simulink model "MLI17"  (R2025a)
settings: Solver=ode45  StartTime=0.0  StopTime=.5  RelTol=1e-3  EnableMultiTasking=on
libraries: spsMosfetLib x12, spsSeriesRLCBranchLib x11, spsVoltageMeasurementLib x10, spsDiodeLib x8, spsControlledCurrentSourceLib x8, spsCurrentMeasurementLib x8, spsParallelRLCLoadLib x1, spspowerguiLib x1
(part 1 of 2)
settings Model: SimulationMode=accelerator  Creator=Indhu  LastModifiedBy=SimuVerity Contributors
settings SolverCC: AlgebraicLoopSolver=TrustRegion
settings DataIOCC: LimitDataPoints=on  SaveFormat=Array  ReturnWorkspaceOutputs=off
settings OptimizationCC: ExpressionDepthLimit=2147483647.0  LifeSpan=inf
settings DebuggingCC: UnderspecifiedInitializationDetection=Classic  MergeDetectMultiDrivingBlocksExec=none  SolverPrmCheckMsg=warning  UnconnectedInputMsg=warning  UnconnectedOutputMsg=warning  UnconnectedLineMsg=warning  StateNameClashWarn=warning  SFUnexpectedBacktrackingDiag=warning  SFNoUnconditionalDefaultTransitionDiag=warning  SFExecutionAtInitializationDiag=none  ArithmeticOperatorsInVariantConditions=warning
settings HardwareCC: ProdBitPerPointer=32.0  ProdBitPerSizeT=32.0  ProdBitPerPtrDiffT=32.0  ProdLargestAtomicFloat=None  ProdIntDivRoundTo=Undefined  ProdEndianess=Unspecified  ProdWordSize=32.0  ProdHWDeviceType=32-bit Generic
settings ModelReferenceCC: PropagateSignalLabelsOutOfModel=off
settings SFSimCC: SimUseLocalCustomCode=off  CustomCodeUndefinedFunction=UseInterfaceOnly
settings RTWCC: RTWUseLocalCustomCode=off  GPUComputeCapability=3.5
settings CodeAppCC: StateflowObjectComments=on
settings GRTTargetCC: TargetLangStandard=C89/C90 (ANSI)
settings ConfigComp: CovMetricSettings=dw  CovSaveCumulativeToWorkspaceVar=on  CovSaveSingleToWorkspaceVar=on  CovExternalEMLEnable=off
settings SimscapeCC: SimscapeNormalizeSystem=off

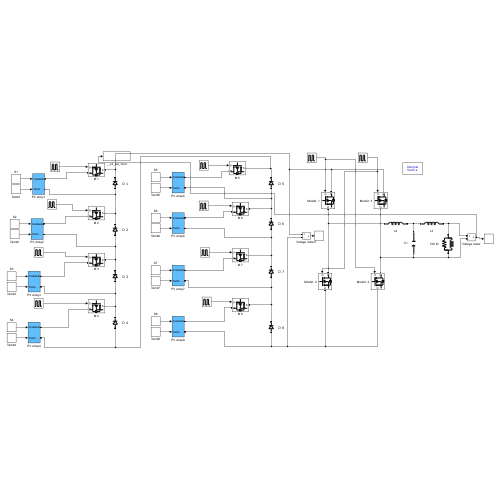
[thumbnail: Simulink's stored preview of the top-level diagram]
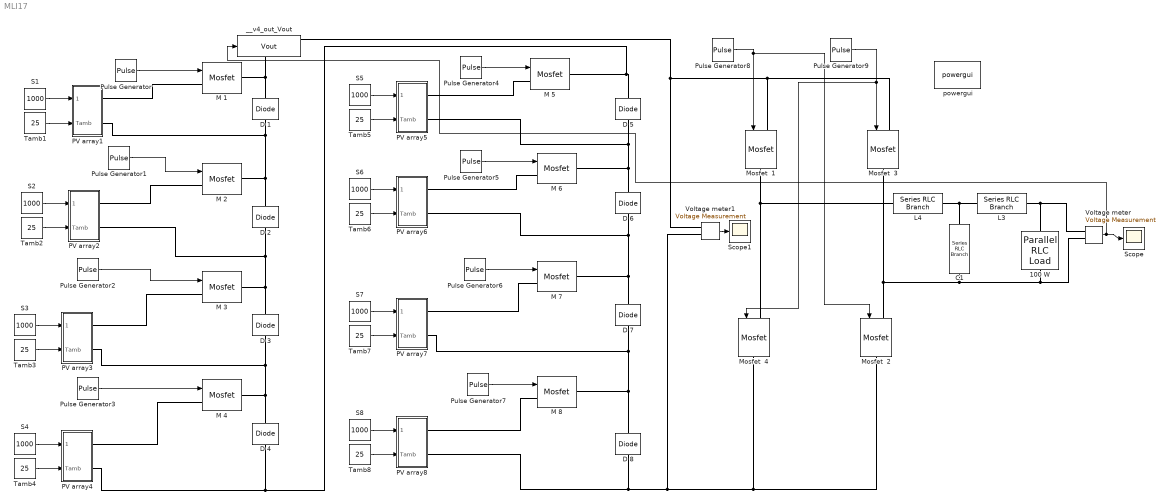
== system MLI17 ==
  100 W : spsParallelRLCLoadLib/Parallel RLC Load  LConnTagsString=a  RConnTagsString=__new0  NominalVoltage=230  NominalFrequency=50  ActivePower=P_load  InductivePower=1  CapacitivePower=0  Setx0=off  InitialVoltage=0  SetiL0=off  InitialCurrent=0  Measurements=None  LoadType=constant Z
      settings: AttributesFormatString=\n  LibrarySourceBlock=sps_lib/Passives/Parallel RLC Load
  C1 : spsSeriesRLCBranchLib/Series RLC Branch  LConnTagsString=__new0  RConnTagsString=__new0  BranchType=C  Resistance=1  Inductance=1e-3  SetiL0=off  InitialCurrent=0  Capacitance=15.5e-5  Setx0=off  InitialVoltage=0  Measurements=None
  D {1..8} (8 alike) : spsDiodeLib/Diode  Ron=0.00001  Lon=0  Vf=0  IC=0  UseSnubber=off  Rs=inf  Cs=0  Measurements=off
  L3 : spsSeriesRLCBranchLib/Series RLC Branch  LConnTagsString=__new0  RConnTagsString=__new0  BranchType=L  Resistance=1  Inductance=0.0499  SetiL0=off  InitialCurrent=0  Capacitance=1e-6  Setx0=off  InitialVoltage=0  Measurements=None
  L4 : spsSeriesRLCBranchLib/Series RLC Branch  LConnTagsString=__new0  RConnTagsString=__new0  BranchType=L  Resistance=1  Inductance=0.04999  SetiL0=off  InitialCurrent=0  Capacitance=1e-6  Setx0=off  InitialVoltage=0  Measurements=None
  M {1..8} (8 alike) : spsMosfetLib/Mosfet  Ron=0.1  Lon=0  Rd=0.01  Vfd=0  IC=0  Rs=1e5  Cs=inf  Measurements=off
  Mosfet  {1..4} (4 alike) : spsMosfetLib/Mosfet  Ron=0.1  Lon=0  Rd=0.01  Vfd=0  IC=0  Rs=1e5  Cs=inf  Measurements=off
  PV array1 : Subsystem
  PV array2 : Subsystem
  PV array3 : Subsystem
  PV array4 : Subsystem
  PV array5 : Subsystem
  PV array6 : Subsystem
  PV array7 : Subsystem
  PV array8 : Subsystem
  Pulse Generator : DiscretePulseGenerator  PulseType=Time based  Period=0.01  PulseWidth=99.999  VectorParams1D=off
  Pulse Generator1 : DiscretePulseGenerator  PulseType=Time based  Period=0.01  PulseWidth=87.5  PhaseDelay=0.000625
  Pulse Generator2 : DiscretePulseGenerator  PulseType=Time based  Period=0.01  PulseWidth=75  PhaseDelay=0.00125
  Pulse Generator3 : DiscretePulseGenerator  PulseType=Time based  Period=0.01  PulseWidth=62.5  PhaseDelay=0.001875
  Pulse Generator4 : DiscretePulseGenerator  PulseType=Time based  Period=0.01  PulseWidth=50  PhaseDelay=0.0025
  Pulse Generator5 : DiscretePulseGenerator  PulseType=Time based  Period=0.01  PulseWidth=37.5  PhaseDelay=0.003125
  Pulse Generator6 : DiscretePulseGenerator  PulseType=Time based  Period=0.01  PulseWidth=25  PhaseDelay=0.00375
  Pulse Generator7 : DiscretePulseGenerator  PulseType=Time based  Period=0.01  PulseWidth=12.5  PhaseDelay=0.004375
  Pulse Generator8 : DiscretePulseGenerator  PulseType=Time based  Period=0.02  PulseWidth=50
  Pulse Generator9 : DiscretePulseGenerator  PulseType=Time based  Period=0.02  PulseWidth=50  PhaseDelay=0.01
  S{1..8} (8 alike) : Constant  Value=1000
  Scope : Scope
      settings: RequirementInfo="{}  %GIDa_4b453156_1c3c_43c0_866a_e0860ec2177e"  Title=17 level output voltage for MCI with LCL filter  ActiveDisplayYMinimum=-225  ActiveDisplayYMaximum=225  DataLoggingMaxPoints=500000000  DataLoggingVariableName=ML
  Scope1 : Scope
      settings: Title="Multilevel DC-DC  output Voltage waveform"
  Tamb{1..8} (8 alike) : Constant  Value=25
  Voltage meter : spsVoltageMeasurementLib/Voltage Measurement  PhasorSimulation=off  OutputType=Complex  PSBequivalent=0
  Voltage meter1 : spsVoltageMeasurementLib/Voltage Measurement  PhasorSimulation=off  OutputType=Complex  PSBequivalent=0
  __v4_out_Vout : ToWorkspace  VariableName=Vout  SaveFormat=Timeseries  SampleTime=-1
  powergui : spspowerguiLib/powergui  Priority=1  SimulationMode=Discrete  SampleTime=50e-6  frequency=60  Iterations=50  frequencyindice=0  Pbase=100e6  ErrMax=1e-4  UnitsV=kV  UnitsW=MW  buscounter=0  FunctionMessages=off  echomessages=off  EnableUseOfTLC=off  CurrentSourceSwitches=off  DisableSnubberDevices=off  DisableRonSwitches=off  DisableVfSwitches=off  DisplayEquations=off  AutomaticDiscreteSolvers=off  SolverType=Tustin  Interpol=off  ExternalGateDelay=off  methode=off  Ts=100  x0status=blocks  SPID=off  SwTol=0  HookPort=off  NonlinearTolerance=1e-4  nMaxIteration=100  ContinueOnMaxIteration=off  RestoreLinks=warning  ResistiveCurrentMeasurement=off  Frange=[0:2:500]  Ylog=off  Xlog=on  ShowGrid=off  save=off  variable=ZData  structure=ML  ZoomFFT=off  StartTime=0.15  cycles=10  DisplayStyle=1  fundamental=50  FreqAxis=off  MaxFrequency=1000  frequencyindicesteady=1  RmsSteady=1  display=off
  wires:
  Voltage meter/1 -> Scope/1, __v4_out_Vout/1
  Pulse Generator/1 -> M 1/1
  Pulse Generator1/1 -> M 2/1
  Pulse Generator2/1 -> M 3/1
  Pulse Generator3/1 -> M 4/1
  Pulse Generator4/1 -> M 5/1
  Pulse Generator5/1 -> M 6/1
  Pulse Generator6/1 -> M 7/1
  Pulse Generator7/1 -> M 8/1
  Pulse Generator8/1 -> Mosfet  2/1, Mosfet  1/1
  Pulse Generator9/1 -> Mosfet  4/1, Mosfet  3/1
  Voltage meter1/1 -> Scope1/1
  Tamb1/1 -> PV array1/2(Tamb)
  S1/1 -> PV array1/1(irradiance)
  Tamb2/1 -> PV array2/2(Tamb)
  S2/1 -> PV array2/1(irradiance)
  Tamb3/1 -> PV array3/2(Tamb)
  S3/1 -> PV array3/1(irradiance)
  Tamb4/1 -> PV array4/2(Tamb)
  S4/1 -> PV array4/1(irradiance)
  Tamb5/1 -> PV array5/2(Tamb)
  S5/1 -> PV array5/1(irradiance)
  Tamb6/1 -> PV array6/2(Tamb)
  S6/1 -> PV array6/1(irradiance)
  Tamb7/1 -> PV array7/2(Tamb)
  S7/1 -> PV array7/1(irradiance)
  Tamb8/1 -> PV array8/2(Tamb)
  S8/1 -> PV array8/1(irradiance)
  connections:
  M 1/LConn1 -- PV array1/RConn1
  D 1/LConn1 -- D 2/RConn1 -- M 2/RConn1 -- PV array1/RConn2
  D 2/LConn1 -- PV array2/RConn2 -- D 3/RConn1 -- M 3/RConn1
  D 3/LConn1 -- D 4/RConn1 -- M 4/RConn1 -- PV array3/RConn2
  M 8/RConn1 -- D 8/RConn1 -- D 7/LConn1 -- PV array7/RConn2
  D 6/LConn1 -- PV array6/RConn2 -- D 7/RConn1 -- M 7/RConn1
  M 6/RConn1 -- D 6/RConn1 -- PV array5/RConn2 -- D 5/LConn1
  M 2/LConn1 -- PV array2/RConn1
  M 3/LConn1 -- PV array3/RConn1
  M 4/LConn1 -- PV array4/RConn1
  D 4/LConn1 -- PV array4/RConn2 -- D 5/RConn1 -- M 5/RConn1
  M 5/LConn1 -- PV array5/RConn1
  M 6/LConn1 -- PV array6/RConn1
  M 7/LConn1 -- PV array7/RConn1
  M 8/LConn1 -- PV array8/RConn1
  Mosfet  4/LConn1 -- L4/LConn1 -- Mosfet  1/RConn1
  Mosfet  3/RConn1 -- C1/RConn1 -- 100 W/RConn1 -- Voltage meter/LConn2 -- Mosfet  2/LConn1
  Voltage meter1/LConn2 -- Mosfet  2/RConn1 -- Mosfet  4/RConn1 -- PV array8/RConn2 -- D 8/LConn1
  Mosfet  1/LConn1 -- Mosfet  3/LConn1 -- Voltage meter1/LConn1 -- M 1/RConn1 -- D 1/RConn1
  C1/LConn1 -- L3/LConn1 -- L4/RConn1
  100 W/LConn1 -- Voltage meter/LConn1 -- L3/RConn1

== system MLI17/PV array1 ==
  irradiance : Inport
  Tamb : Inport  Port=2
  4700uF : spsSeriesRLCBranchLib/Series RLC Branch  LConnTagsString=__new0  RConnTagsString=__new0  BranchType=C  Resistance=1  Inductance=5e-03  SetiL0=off  InitialCurrent=0  Capacitance=4700e-6  Setx0=off  InitialVoltage=0  Measurements=None
  CCS : spsControlledCurrentSourceLib/Controlled Current Source  Initialize=on  Source_Type=AC  Amplitude=0  Phase=0  Frequency=0  Measurements=None
  CM : spsCurrentMeasurementLib/Current Measurement  PhasorSimulation=off  OutputType=Complex  PSBequivalent=0
  Im : Constant  Value=10
  Isc : Constant  Value=12
  Saturation : Saturate  UpperLimit=100  LowerLimit=0
  Saturation1 : Saturate  UpperLimit=4  LowerLimit=0
  Subsystem1 : Subsystem
  Tref : Constant  Value=55
  VM1 : spsVoltageMeasurementLib/Voltage Measurement  PhasorSimulation=off  OutputType=Complex  PSBequivalent=0
  Vm : Constant  Value=28
  Voc : Constant  Value=28.75
  + : PMIOPort  Tag=PMCPort  Side=Right
  - : PMIOPort  Tag=PMCPort  Port=2  Side=Right
  wires:
  Isc/1 -> Subsystem1/4(Isc)
  Im/1 -> Subsystem1/6(Im)
  Voc/1 -> Subsystem1/5(Voc)
  Vm/1 -> Subsystem1/7(Vm)
  irradiance/1 -> Subsystem1/2(S)
  Tamb/1 -> Subsystem1/3(Tamb)
  Saturation/1 -> Subsystem1/1(Vpv)
  VM1/1 -> Saturation/1
  Tref/1 -> Subsystem1/8(Tref)
  Subsystem1/1(Ipv) -> Saturation1/1
  Saturation1/1 -> CCS/1
  connections:
  CCS/RConn1 -- CM/LConn1
  +/RConn1 -- CM/RConn1 -- VM1/LConn1 -- 4700uF/LConn1
  -/RConn1 -- CCS/LConn1 -- VM1/LConn2 -- 4700uF/RConn1

== system MLI17/PV array2 ==
  irradiance : Inport
  Tamb : Inport  Port=2
  4700uF : spsSeriesRLCBranchLib/Series RLC Branch  LConnTagsString=__new0  RConnTagsString=__new0  BranchType=C  Resistance=1  Inductance=5e-03  SetiL0=off  InitialCurrent=0  Capacitance=4700e-6  Setx0=off  InitialVoltage=0  Measurements=None
  CCS : spsControlledCurrentSourceLib/Controlled Current Source  Initialize=on  Source_Type=AC  Amplitude=0  Phase=0  Frequency=0  Measurements=None
  CM : spsCurrentMeasurementLib/Current Measurement  PhasorSimulation=off  OutputType=Complex  PSBequivalent=0
  Im : Constant  Value=10
  Isc : Constant  Value=12
  Saturation : Saturate  UpperLimit=100  LowerLimit=0
  Saturation1 : Saturate  UpperLimit=4  LowerLimit=0
  Subsystem1 : Subsystem
  Tref : Constant  Value=55
  VM1 : spsVoltageMeasurementLib/Voltage Measurement  PhasorSimulation=off  OutputType=Complex  PSBequivalent=0
  Vm : Constant  Value=28
  Voc : Constant  Value=28.75
  + : PMIOPort  Tag=PMCPort  Side=Right
  - : PMIOPort  Tag=PMCPort  Port=2  Side=Right
  wires:
  Saturation1/1 -> CCS/1
  Subsystem1/1(Ipv) -> Saturation1/1
  Tref/1 -> Subsystem1/8(Tref)
  VM1/1 -> Saturation/1
  Saturation/1 -> Subsystem1/1(Vpv)
  Tamb/1 -> Subsystem1/3(Tamb)
  irradiance/1 -> Subsystem1/2(S)
  Vm/1 -> Subsystem1/7(Vm)
  Voc/1 -> Subsystem1/5(Voc)
  Im/1 -> Subsystem1/6(Im)
  Isc/1 -> Subsystem1/4(Isc)
  connections:
  4700uF/RConn1 -- VM1/LConn2 -- CCS/LConn1 -- -/RConn1
  4700uF/LConn1 -- VM1/LConn1 -- CM/RConn1 -- +/RConn1
  CCS/RConn1 -- CM/LConn1

== system MLI17/PV array3 ==
  irradiance : Inport
  Tamb : Inport  Port=2
  4700uF : spsSeriesRLCBranchLib/Series RLC Branch  LConnTagsString=__new0  RConnTagsString=__new0  BranchType=C  Resistance=1  Inductance=5e-03  SetiL0=off  InitialCurrent=0  Capacitance=4700e-6  Setx0=off  InitialVoltage=0  Measurements=None
  CCS : spsControlledCurrentSourceLib/Controlled Current Source  Initialize=on  Source_Type=AC  Amplitude=0  Phase=0  Frequency=0  Measurements=None
  CM : spsCurrentMeasurementLib/Current Measurement  PhasorSimulation=off  OutputType=Complex  PSBequivalent=0
  Im : Constant  Value=10
  Isc : Constant  Value=12
  Saturation : Saturate  UpperLimit=100  LowerLimit=0
  Saturation1 : Saturate  UpperLimit=4  LowerLimit=0
  Subsystem1 : Subsystem
  Tref : Constant  Value=55
  VM1 : spsVoltageMeasurementLib/Voltage Measurement  PhasorSimulation=off  OutputType=Complex  PSBequivalent=0
  Vm : Constant  Value=28
  Voc : Constant  Value=28.75
  + : PMIOPort  Tag=PMCPort  Side=Right
  - : PMIOPort  Tag=PMCPort  Port=2  Side=Right
  wires:
  Isc/1 -> Subsystem1/4(Isc)
  Im/1 -> Subsystem1/6(Im)
  Voc/1 -> Subsystem1/5(Voc)
  Vm/1 -> Subsystem1/7(Vm)
  irradiance/1 -> Subsystem1/2(S)
  Tamb/1 -> Subsystem1/3(Tamb)
  Saturation/1 -> Subsystem1/1(Vpv)
  VM1/1 -> Saturation/1
  Tref/1 -> Subsystem1/8(Tref)
  Subsystem1/1(Ipv) -> Saturation1/1
  Saturation1/1 -> CCS/1
  connections:
  CCS/RConn1 -- CM/LConn1
  +/RConn1 -- CM/RConn1 -- VM1/LConn1 -- 4700uF/LConn1
  -/RConn1 -- CCS/LConn1 -- VM1/LConn2 -- 4700uF/RConn1

== system MLI17/PV array4 ==
  irradiance : Inport
  Tamb : Inport  Port=2
  4700uF : spsSeriesRLCBranchLib/Series RLC Branch  LConnTagsString=__new0  RConnTagsString=__new0  BranchType=C  Resistance=1  Inductance=5e-03  SetiL0=off  InitialCurrent=0  Capacitance=4700e-6  Setx0=off  InitialVoltage=0  Measurements=None
  CCS : spsControlledCurrentSourceLib/Controlled Current Source  Initialize=on  Source_Type=AC  Amplitude=0  Phase=0  Frequency=0  Measurements=None
  CM : spsCurrentMeasurementLib/Current Measurement  PhasorSimulation=off  OutputType=Complex  PSBequivalent=0
  Im : Constant  Value=10
  Isc : Constant  Value=12
  Saturation : Saturate  UpperLimit=100  LowerLimit=0
  Saturation1 : Saturate  UpperLimit=4  LowerLimit=0
  Subsystem1 : Subsystem
  Tref : Constant  Value=55
  VM1 : spsVoltageMeasurementLib/Voltage Measurement  PhasorSimulation=off  OutputType=Complex  PSBequivalent=0
  Vm : Constant  Value=28
  Voc : Constant  Value=28.75
  + : PMIOPort  Tag=PMCPort  Side=Right
  - : PMIOPort  Tag=PMCPort  Port=2  Side=Right
  wires:
  Saturation1/1 -> CCS/1
  Subsystem1/1(Ipv) -> Saturation1/1
  Tref/1 -> Subsystem1/8(Tref)
  VM1/1 -> Saturation/1
  Saturation/1 -> Subsystem1/1(Vpv)
  Tamb/1 -> Subsystem1/3(Tamb)
  irradiance/1 -> Subsystem1/2(S)
  Vm/1 -> Subsystem1/7(Vm)
  Voc/1 -> Subsystem1/5(Voc)
  Im/1 -> Subsystem1/6(Im)
  Isc/1 -> Subsystem1/4(Isc)
  connections:
  4700uF/RConn1 -- VM1/LConn2 -- CCS/LConn1 -- -/RConn1
  4700uF/LConn1 -- VM1/LConn1 -- CM/RConn1 -- +/RConn1
  CCS/RConn1 -- CM/LConn1

== system MLI17/PV array5 ==
  irradiance : Inport
  Tamb : Inport  Port=2
  4700uF : spsSeriesRLCBranchLib/Series RLC Branch  LConnTagsString=__new0  RConnTagsString=__new0  BranchType=C  Resistance=1  Inductance=5e-03  SetiL0=off  InitialCurrent=0  Capacitance=4700e-6  Setx0=off  InitialVoltage=0  Measurements=None
  CCS : spsControlledCurrentSourceLib/Controlled Current Source  Initialize=on  Source_Type=AC  Amplitude=0  Phase=0  Frequency=0  Measurements=None
  CM : spsCurrentMeasurementLib/Current Measurement  PhasorSimulation=off  OutputType=Complex  PSBequivalent=0
  Im : Constant  Value=10
  Isc : Constant  Value=12
  Saturation : Saturate  UpperLimit=100  LowerLimit=0
  Saturation1 : Saturate  UpperLimit=4  LowerLimit=0
  Subsystem1 : Subsystem
  Tref : Constant  Value=55
  VM1 : spsVoltageMeasurementLib/Voltage Measurement  PhasorSimulation=off  OutputType=Complex  PSBequivalent=0
  Vm : Constant  Value=28
  Voc : Constant  Value=28.75
  + : PMIOPort  Tag=PMCPort  Side=Right
  - : PMIOPort  Tag=PMCPort  Port=2  Side=Right
  wires:
  Isc/1 -> Subsystem1/4(Isc)
  Im/1 -> Subsystem1/6(Im)
  Voc/1 -> Subsystem1/5(Voc)
  Vm/1 -> Subsystem1/7(Vm)
  irradiance/1 -> Subsystem1/2(S)
  Tamb/1 -> Subsystem1/3(Tamb)
  Saturation/1 -> Subsystem1/1(Vpv)
  VM1/1 -> Saturation/1
  Tref/1 -> Subsystem1/8(Tref)
  Subsystem1/1(Ipv) -> Saturation1/1
  Saturation1/1 -> CCS/1
  connections:
  CCS/RConn1 -- CM/LConn1
  +/RConn1 -- CM/RConn1 -- VM1/LConn1 -- 4700uF/LConn1
  -/RConn1 -- CCS/LConn1 -- VM1/LConn2 -- 4700uF/RConn1

== system MLI17/PV array6 ==
  irradiance : Inport
  Tamb : Inport  Port=2
  4700uF : spsSeriesRLCBranchLib/Series RLC Branch  LConnTagsString=__new0  RConnTagsString=__new0  BranchType=C  Resistance=1  Inductance=5e-03  SetiL0=off  InitialCurrent=0  Capacitance=4700e-6  Setx0=off  InitialVoltage=0  Measurements=None
  CCS : spsControlledCurrentSourceLib/Controlled Current Source  Initialize=on  Source_Type=AC  Amplitude=0  Phase=0  Frequency=0  Measurements=None
  CM : spsCurrentMeasurementLib/Current Measurement  PhasorSimulation=off  OutputType=Complex  PSBequivalent=0
  Im : Constant  Value=10
  Isc : Constant  Value=12
  Saturation : Saturate  UpperLimit=100  LowerLimit=0
  Saturation1 : Saturate  UpperLimit=4  LowerLimit=0
  Subsystem1 : Subsystem
  Tref : Constant  Value=55
  VM1 : spsVoltageMeasurementLib/Voltage Measurement  PhasorSimulation=off  OutputType=Complex  PSBequivalent=0
  Vm : Constant  Value=28
  Voc : Constant  Value=28.75
  + : PMIOPort  Tag=PMCPort  Side=Right
  - : PMIOPort  Tag=PMCPort  Port=2  Side=Right
  wires:
  Saturation1/1 -> CCS/1
  Subsystem1/1(Ipv) -> Saturation1/1
  Tref/1 -> Subsystem1/8(Tref)
  VM1/1 -> Saturation/1
  Saturation/1 -> Subsystem1/1(Vpv)
  Tamb/1 -> Subsystem1/3(Tamb)
  irradiance/1 -> Subsystem1/2(S)
  Vm/1 -> Subsystem1/7(Vm)
  Voc/1 -> Subsystem1/5(Voc)
  Im/1 -> Subsystem1/6(Im)
  Isc/1 -> Subsystem1/4(Isc)
  connections:
  4700uF/RConn1 -- VM1/LConn2 -- CCS/LConn1 -- -/RConn1
  4700uF/LConn1 -- VM1/LConn1 -- CM/RConn1 -- +/RConn1
  CCS/RConn1 -- CM/LConn1

== system MLI17/PV array7 ==
  irradiance : Inport
  Tamb : Inport  Port=2
  4700uF : spsSeriesRLCBranchLib/Series RLC Branch  LConnTagsString=__new0  RConnTagsString=__new0  BranchType=C  Resistance=1  Inductance=5e-03  SetiL0=off  InitialCurrent=0  Capacitance=4700e-6  Setx0=off  InitialVoltage=0  Measurements=None
  CCS : spsControlledCurrentSourceLib/Controlled Current Source  Initialize=on  Source_Type=AC  Amplitude=0  Phase=0  Frequency=0  Measurements=None
  CM : spsCurrentMeasurementLib/Current Measurement  PhasorSimulation=off  OutputType=Complex  PSBequivalent=0
  Im : Constant  Value=10
  Isc : Constant  Value=12
  Saturation : Saturate  UpperLimit=100  LowerLimit=0
  Saturation1 : Saturate  UpperLimit=4  LowerLimit=0
  Subsystem1 : Subsystem
  Tref : Constant  Value=55
  VM1 : spsVoltageMeasurementLib/Voltage Measurement  PhasorSimulation=off  OutputType=Complex  PSBequivalent=0
  Vm : Constant  Value=28
  Voc : Constant  Value=28.75
  + : PMIOPort  Tag=PMCPort  Side=Right
  - : PMIOPort  Tag=PMCPort  Port=2  Side=Right
  wires:
  Isc/1 -> Subsystem1/4(Isc)
  Im/1 -> Subsystem1/6(Im)
  Voc/1 -> Subsystem1/5(Voc)
  Vm/1 -> Subsystem1/7(Vm)
  irradiance/1 -> Subsystem1/2(S)
  Tamb/1 -> Subsystem1/3(Tamb)
  Saturation/1 -> Subsystem1/1(Vpv)
  VM1/1 -> Saturation/1
  Tref/1 -> Subsystem1/8(Tref)
  Subsystem1/1(Ipv) -> Saturation1/1
  Saturation1/1 -> CCS/1
  connections:
  CCS/RConn1 -- CM/LConn1
  +/RConn1 -- CM/RConn1 -- VM1/LConn1 -- 4700uF/LConn1
  -/RConn1 -- CCS/LConn1 -- VM1/LConn2 -- 4700uF/RConn1

== system MLI17/PV array8 ==
  irradiance : Inport
  Tamb : Inport  Port=2
  4700uF : spsSeriesRLCBranchLib/Series RLC Branch  LConnTagsString=__new0  RConnTagsString=__new0  BranchType=C  Resistance=1  Inductance=5e-03  SetiL0=off  InitialCurrent=0  Capacitance=4700e-6  Setx0=off  InitialVoltage=0  Measurements=None
  CCS : spsControlledCurrentSourceLib/Controlled Current Source  Initialize=on  Source_Type=AC  Amplitude=0  Phase=0  Frequency=0  Measurements=None
  CM : spsCurrentMeasurementLib/Current Measurement  PhasorSimulation=off  OutputType=Complex  PSBequivalent=0
  Im : Constant  Value=10
  Isc : Constant  Value=12
  Saturation : Saturate  UpperLimit=100  LowerLimit=0
  Saturation1 : Saturate  UpperLimit=4  LowerLimit=0
  Subsystem1 : Subsystem
  Tref : Constant  Value=55
  VM1 : spsVoltageMeasurementLib/Voltage Measurement  PhasorSimulation=off  OutputType=Complex  PSBequivalent=0
  Vm : Constant  Value=28
  Voc : Constant  Value=28.75
  + : PMIOPort  Tag=PMCPort  Side=Right
  - : PMIOPort  Tag=PMCPort  Port=2  Side=Right
  wires:
  Saturation1/1 -> CCS/1
  Subsystem1/1(Ipv) -> Saturation1/1
  Tref/1 -> Subsystem1/8(Tref)
  VM1/1 -> Saturation/1
  Saturation/1 -> Subsystem1/1(Vpv)
  Tamb/1 -> Subsystem1/3(Tamb)
  irradiance/1 -> Subsystem1/2(S)
  Vm/1 -> Subsystem1/7(Vm)
  Voc/1 -> Subsystem1/5(Voc)
  Im/1 -> Subsystem1/6(Im)
  Isc/1 -> Subsystem1/4(Isc)
  connections:
  4700uF/RConn1 -- VM1/LConn2 -- CCS/LConn1 -- -/RConn1
  4700uF/LConn1 -- VM1/LConn1 -- CM/RConn1 -- +/RConn1
  CCS/RConn1 -- CM/LConn1

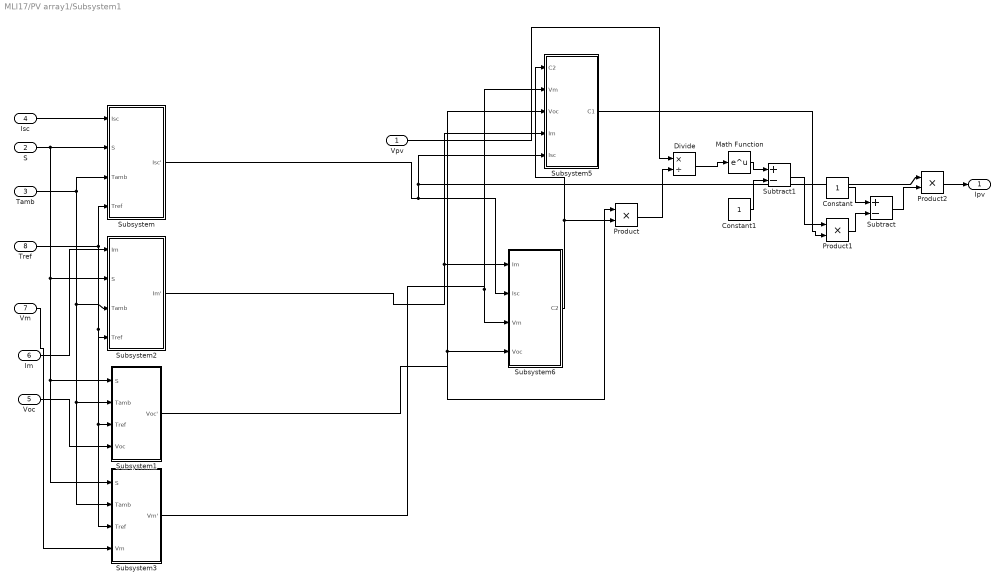
== system MLI17/PV array1/Subsystem1 ==
  Vpv : Inport
  S : Inport  Port=2
  Tamb : Inport  Port=3
  Isc : Inport  Port=4
  Voc : Inport  Port=5
  Im : Inport  Port=6
  Vm : Inport  Port=7
  Tref : Inport  Port=8
  Constant : Constant
  Constant1 : Constant
  Divide : Product  Inputs=*/
  Math Function : Math  SignedPower=on
  Product : Product  RndMeth=Zero
  Product1 : Product  RndMeth=Zero
  Product2 : Product  RndMeth=Zero
  Subsystem : Subsystem
  Subsystem1 : Subsystem
  Subsystem2 : Subsystem
  Subsystem3 : Subsystem
  Subsystem5 : Subsystem
  Subsystem6 : Subsystem
  Subtract : Sum  Inputs=+-
  Subtract1 : Sum  Inputs=+-
  Ipv : Outport
  wires:
  Product/1 -> Divide/2
  Constant/1 -> Subtract/1
  Product1/1 -> Subtract/2
  Subtract/1 -> Product2/2
  Product2/1 -> Ipv/1
  Divide/1 -> Math Function/1
  Math Function/1 -> Subtract1/1
  Constant1/1 -> Subtract1/2
  Subtract1/1 -> Product1/1
  Subsystem2/1(Im') -> Subsystem6/1(Im), Subsystem5/4(Im)
  Subsystem/1(Isc') -> Subsystem6/2(Isc), Product2/1, Subsystem5/5(Isc)
  Subsystem1/1(Voc') -> Product/1, Subsystem5/3(Voc), Subsystem6/4(Voc)
  Subsystem3/1(Vm') -> Subsystem5/2(Vm), Subsystem6/3(Vm)
  Subsystem6/1(C2) -> Subsystem5/1(C2), Product/2
  Vpv/1 -> Divide/1
  Subsystem5/1(C1) -> Product1/2
  Isc/1 -> Subsystem/1(Isc)
  S/1 -> Subsystem1/1(S), Subsystem3/1(S), Subsystem2/2(S), Subsystem/2(S)
  Tamb/1 -> Subsystem1/2(Tamb), Subsystem3/2(Tamb), Subsystem2/3(Tamb), Subsystem/3(Tamb)
  Tref/1 -> Subsystem1/3(Tref), Subsystem3/3(Tref), Subsystem2/4(Tref), Subsystem/4(Tref)
  Im/1 -> Subsystem2/1(Im)
  Voc/1 -> Subsystem1/4(Voc)
  Vm/1 -> Subsystem3/4(Vm)

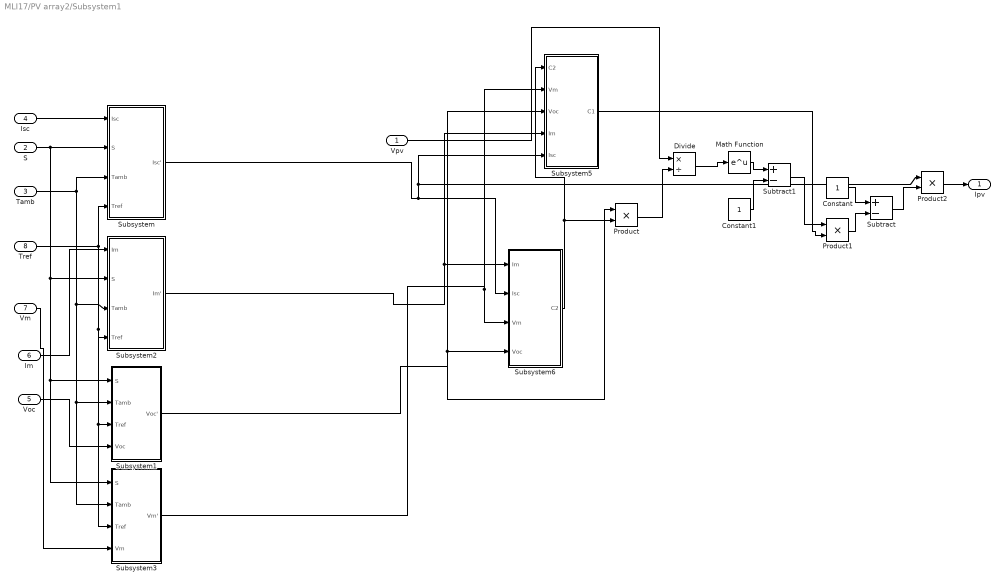
== system MLI17/PV array2/Subsystem1 ==
  Vpv : Inport
  S : Inport  Port=2
  Tamb : Inport  Port=3
  Isc : Inport  Port=4
  Voc : Inport  Port=5
  Im : Inport  Port=6
  Vm : Inport  Port=7
  Tref : Inport  Port=8
  Constant : Constant
  Constant1 : Constant
  Divide : Product  Inputs=*/
  Math Function : Math  SignedPower=on
  Product : Product  RndMeth=Zero
  Product1 : Product  RndMeth=Zero
  Product2 : Product  RndMeth=Zero
  Subsystem : Subsystem
  Subsystem1 : Subsystem
  Subsystem2 : Subsystem
  Subsystem3 : Subsystem
  Subsystem5 : Subsystem
  Subsystem6 : Subsystem
  Subtract : Sum  Inputs=+-
  Subtract1 : Sum  Inputs=+-
  Ipv : Outport
  wires:
  Vm/1 -> Subsystem3/4(Vm)
  Voc/1 -> Subsystem1/4(Voc)
  Im/1 -> Subsystem2/1(Im)
  Tref/1 -> Subsystem/4(Tref), Subsystem2/4(Tref), Subsystem3/3(Tref), Subsystem1/3(Tref)
  Tamb/1 -> Subsystem/3(Tamb), Subsystem2/3(Tamb), Subsystem3/2(Tamb), Subsystem1/2(Tamb)
  S/1 -> Subsystem/2(S), Subsystem2/2(S), Subsystem3/1(S), Subsystem1/1(S)
  Isc/1 -> Subsystem/1(Isc)
  Subsystem5/1(C1) -> Product1/2
  Vpv/1 -> Divide/1
  Subsystem6/1(C2) -> Product/2, Subsystem5/1(C2)
  Subsystem3/1(Vm') -> Subsystem6/3(Vm), Subsystem5/2(Vm)
  Subsystem1/1(Voc') -> Subsystem6/4(Voc), Subsystem5/3(Voc), Product/1
  Subsystem/1(Isc') -> Subsystem5/5(Isc), Product2/1, Subsystem6/2(Isc)
  Subsystem2/1(Im') -> Subsystem5/4(Im), Subsystem6/1(Im)
  Subtract1/1 -> Product1/1
  Constant1/1 -> Subtract1/2
  Math Function/1 -> Subtract1/1
  Divide/1 -> Math Function/1
  Product2/1 -> Ipv/1
  Subtract/1 -> Product2/2
  Product1/1 -> Subtract/2
  Constant/1 -> Subtract/1
  Product/1 -> Divide/2

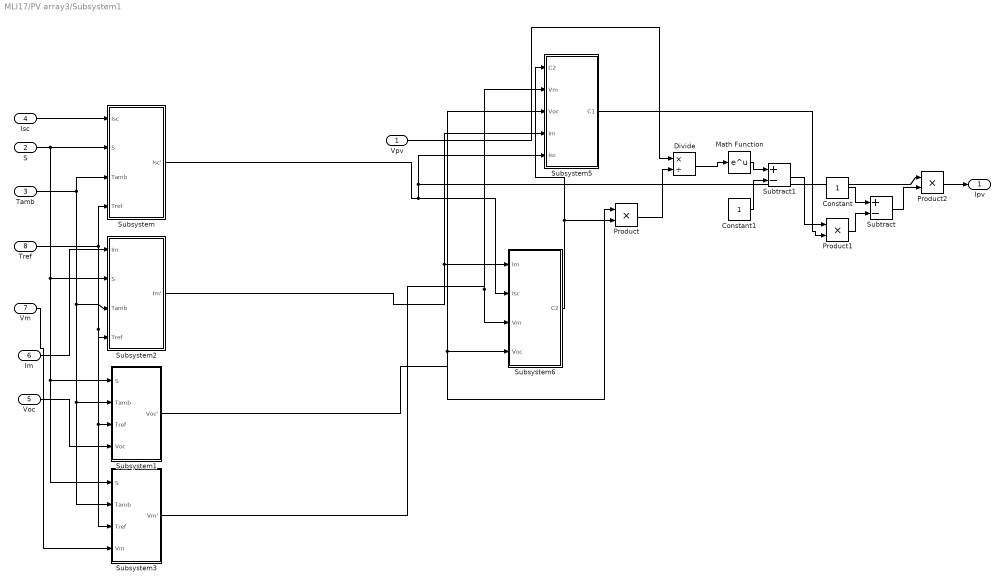
== system MLI17/PV array3/Subsystem1 ==
  Vpv : Inport
  S : Inport  Port=2
  Tamb : Inport  Port=3
  Isc : Inport  Port=4
  Voc : Inport  Port=5
  Im : Inport  Port=6
  Vm : Inport  Port=7
  Tref : Inport  Port=8
  Constant : Constant
  Constant1 : Constant
  Divide : Product  Inputs=*/
  Math Function : Math  SignedPower=on
  Product : Product  RndMeth=Zero
  Product1 : Product  RndMeth=Zero
  Product2 : Product  RndMeth=Zero
  Subsystem : Subsystem
  Subsystem1 : Subsystem
  Subsystem2 : Subsystem
  Subsystem3 : Subsystem
  Subsystem5 : Subsystem
  Subsystem6 : Subsystem
  Subtract : Sum  Inputs=+-
  Subtract1 : Sum  Inputs=+-
  Ipv : Outport
  wires:
  Product/1 -> Divide/2
  Constant/1 -> Subtract/1
  Product1/1 -> Subtract/2
  Subtract/1 -> Product2/2
  Product2/1 -> Ipv/1
  Divide/1 -> Math Function/1
  Math Function/1 -> Subtract1/1
  Constant1/1 -> Subtract1/2
  Subtract1/1 -> Product1/1
  Subsystem2/1(Im') -> Subsystem6/1(Im), Subsystem5/4(Im)
  Subsystem/1(Isc') -> Subsystem6/2(Isc), Product2/1, Subsystem5/5(Isc)
  Subsystem1/1(Voc') -> Product/1, Subsystem5/3(Voc), Subsystem6/4(Voc)
  Subsystem3/1(Vm') -> Subsystem5/2(Vm), Subsystem6/3(Vm)
  Subsystem6/1(C2) -> Subsystem5/1(C2), Product/2
  Vpv/1 -> Divide/1
  Subsystem5/1(C1) -> Product1/2
  Isc/1 -> Subsystem/1(Isc)
  S/1 -> Subsystem1/1(S), Subsystem3/1(S), Subsystem2/2(S), Subsystem/2(S)
  Tamb/1 -> Subsystem1/2(Tamb), Subsystem3/2(Tamb), Subsystem2/3(Tamb), Subsystem/3(Tamb)
  Tref/1 -> Subsystem1/3(Tref), Subsystem3/3(Tref), Subsystem2/4(Tref), Subsystem/4(Tref)
  Im/1 -> Subsystem2/1(Im)
  Voc/1 -> Subsystem1/4(Voc)
  Vm/1 -> Subsystem3/4(Vm)

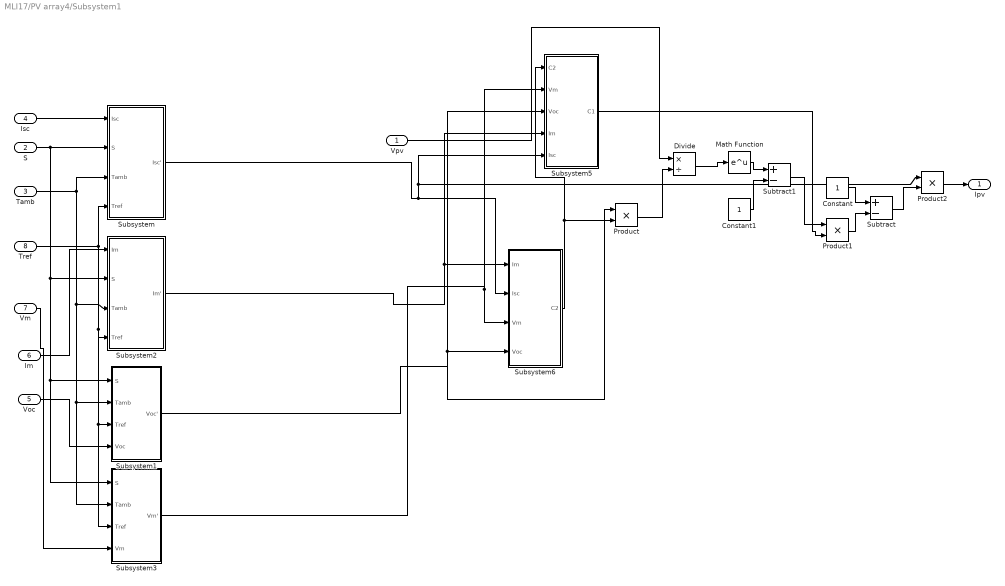
== system MLI17/PV array4/Subsystem1 ==
  Vpv : Inport
  S : Inport  Port=2
  Tamb : Inport  Port=3
  Isc : Inport  Port=4
  Voc : Inport  Port=5
  Im : Inport  Port=6
  Vm : Inport  Port=7
  Tref : Inport  Port=8
  Constant : Constant
  Constant1 : Constant
  Divide : Product  Inputs=*/
  Math Function : Math  SignedPower=on
  Product : Product  RndMeth=Zero
  Product1 : Product  RndMeth=Zero
  Product2 : Product  RndMeth=Zero
  Subsystem : Subsystem
  Subsystem1 : Subsystem
  Subsystem2 : Subsystem
  Subsystem3 : Subsystem
  Subsystem5 : Subsystem
  Subsystem6 : Subsystem
  Subtract : Sum  Inputs=+-
  Subtract1 : Sum  Inputs=+-
  Ipv : Outport
  wires:
  Vm/1 -> Subsystem3/4(Vm)
  Voc/1 -> Subsystem1/4(Voc)
  Im/1 -> Subsystem2/1(Im)
  Tref/1 -> Subsystem/4(Tref), Subsystem2/4(Tref), Subsystem3/3(Tref), Subsystem1/3(Tref)
  Tamb/1 -> Subsystem/3(Tamb), Subsystem2/3(Tamb), Subsystem3/2(Tamb), Subsystem1/2(Tamb)
  S/1 -> Subsystem/2(S), Subsystem2/2(S), Subsystem3/1(S), Subsystem1/1(S)
  Isc/1 -> Subsystem/1(Isc)
  Subsystem5/1(C1) -> Product1/2
  Vpv/1 -> Divide/1
  Subsystem6/1(C2) -> Product/2, Subsystem5/1(C2)
  Subsystem3/1(Vm') -> Subsystem6/3(Vm), Subsystem5/2(Vm)
  Subsystem1/1(Voc') -> Subsystem6/4(Voc), Subsystem5/3(Voc), Product/1
  Subsystem/1(Isc') -> Subsystem5/5(Isc), Product2/1, Subsystem6/2(Isc)
  Subsystem2/1(Im') -> Subsystem5/4(Im), Subsystem6/1(Im)
  Subtract1/1 -> Product1/1
  Constant1/1 -> Subtract1/2
  Math Function/1 -> Subtract1/1
  Divide/1 -> Math Function/1
  Product2/1 -> Ipv/1
  Subtract/1 -> Product2/2
  Product1/1 -> Subtract/2
  Constant/1 -> Subtract/1
  Product/1 -> Divide/2

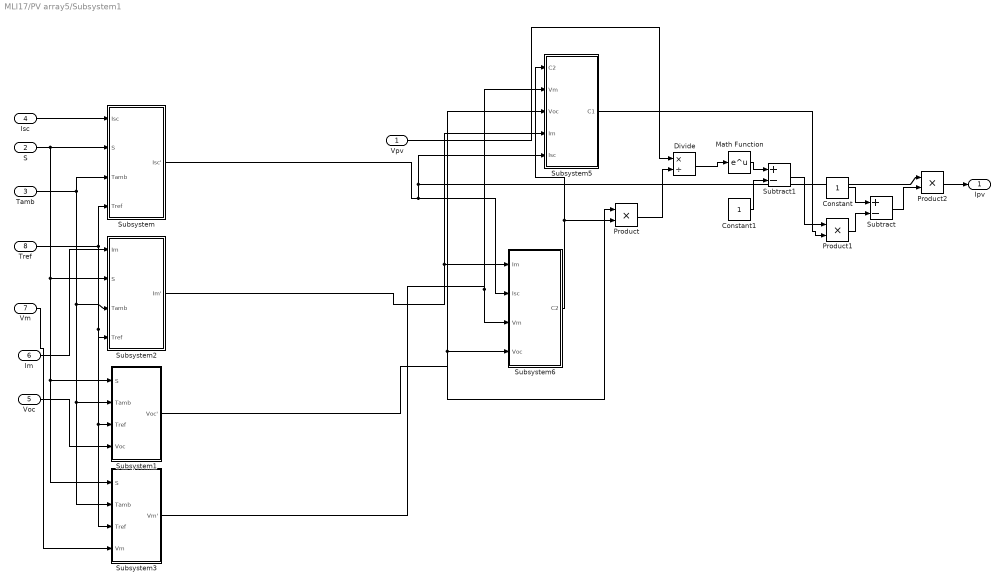
== system MLI17/PV array5/Subsystem1 ==
  Vpv : Inport
  S : Inport  Port=2
  Tamb : Inport  Port=3
  Isc : Inport  Port=4
  Voc : Inport  Port=5
  Im : Inport  Port=6
  Vm : Inport  Port=7
  Tref : Inport  Port=8
  Constant : Constant
  Constant1 : Constant
  Divide : Product  Inputs=*/
  Math Function : Math  SignedPower=on
  Product : Product  RndMeth=Zero
  Product1 : Product  RndMeth=Zero
  Product2 : Product  RndMeth=Zero
  Subsystem : Subsystem
  Subsystem1 : Subsystem
  Subsystem2 : Subsystem
  Subsystem3 : Subsystem
  Subsystem5 : Subsystem
  Subsystem6 : Subsystem
  Subtract : Sum  Inputs=+-
  Subtract1 : Sum  Inputs=+-
  Ipv : Outport
  wires:
  Product/1 -> Divide/2
  Constant/1 -> Subtract/1
  Product1/1 -> Subtract/2
  Subtract/1 -> Product2/2
  Product2/1 -> Ipv/1
  Divide/1 -> Math Function/1
  Math Function/1 -> Subtract1/1
  Constant1/1 -> Subtract1/2
  Subtract1/1 -> Product1/1
  Subsystem2/1(Im') -> Subsystem6/1(Im), Subsystem5/4(Im)
  Subsystem/1(Isc') -> Subsystem6/2(Isc), Product2/1, Subsystem5/5(Isc)
  Subsystem1/1(Voc') -> Product/1, Subsystem5/3(Voc), Subsystem6/4(Voc)
  Subsystem3/1(Vm') -> Subsystem5/2(Vm), Subsystem6/3(Vm)
  Subsystem6/1(C2) -> Subsystem5/1(C2), Product/2
  Vpv/1 -> Divide/1
  Subsystem5/1(C1) -> Product1/2
  Isc/1 -> Subsystem/1(Isc)
  S/1 -> Subsystem1/1(S), Subsystem3/1(S), Subsystem2/2(S), Subsystem/2(S)
  Tamb/1 -> Subsystem1/2(Tamb), Subsystem3/2(Tamb), Subsystem2/3(Tamb), Subsystem/3(Tamb)
  Tref/1 -> Subsystem1/3(Tref), Subsystem3/3(Tref), Subsystem2/4(Tref), Subsystem/4(Tref)
  Im/1 -> Subsystem2/1(Im)
  Voc/1 -> Subsystem1/4(Voc)
  Vm/1 -> Subsystem3/4(Vm)

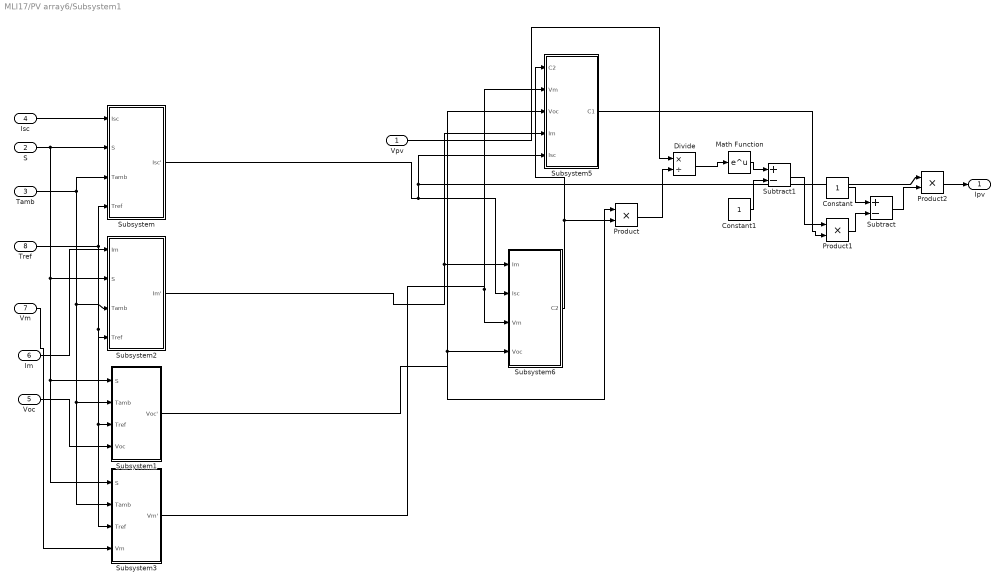
== system MLI17/PV array6/Subsystem1 ==
  Vpv : Inport
  S : Inport  Port=2
  Tamb : Inport  Port=3
  Isc : Inport  Port=4
  Voc : Inport  Port=5
  Im : Inport  Port=6
  Vm : Inport  Port=7
  Tref : Inport  Port=8
  Constant : Constant
  Constant1 : Constant
  Divide : Product  Inputs=*/
  Math Function : Math  SignedPower=on
  Product : Product  RndMeth=Zero
  Product1 : Product  RndMeth=Zero
  Product2 : Product  RndMeth=Zero
  Subsystem : Subsystem
  Subsystem1 : Subsystem
  Subsystem2 : Subsystem
  Subsystem3 : Subsystem
  Subsystem5 : Subsystem
  Subsystem6 : Subsystem
  Subtract : Sum  Inputs=+-
  Subtract1 : Sum  Inputs=+-
  Ipv : Outport
  wires:
  Vm/1 -> Subsystem3/4(Vm)
  Voc/1 -> Subsystem1/4(Voc)
  Im/1 -> Subsystem2/1(Im)
  Tref/1 -> Subsystem/4(Tref), Subsystem2/4(Tref), Subsystem3/3(Tref), Subsystem1/3(Tref)
  Tamb/1 -> Subsystem/3(Tamb), Subsystem2/3(Tamb), Subsystem3/2(Tamb), Subsystem1/2(Tamb)
  S/1 -> Subsystem/2(S), Subsystem2/2(S), Subsystem3/1(S), Subsystem1/1(S)
  Isc/1 -> Subsystem/1(Isc)
  Subsystem5/1(C1) -> Product1/2
  Vpv/1 -> Divide/1
  Subsystem6/1(C2) -> Product/2, Subsystem5/1(C2)
  Subsystem3/1(Vm') -> Subsystem6/3(Vm), Subsystem5/2(Vm)
  Subsystem1/1(Voc') -> Subsystem6/4(Voc), Subsystem5/3(Voc), Product/1
  Subsystem/1(Isc') -> Subsystem5/5(Isc), Product2/1, Subsystem6/2(Isc)
  Subsystem2/1(Im') -> Subsystem5/4(Im), Subsystem6/1(Im)
  Subtract1/1 -> Product1/1
  Constant1/1 -> Subtract1/2
  Math Function/1 -> Subtract1/1
  Divide/1 -> Math Function/1
  Product2/1 -> Ipv/1
  Subtract/1 -> Product2/2
  Product1/1 -> Subtract/2
  Constant/1 -> Subtract/1
  Product/1 -> Divide/2

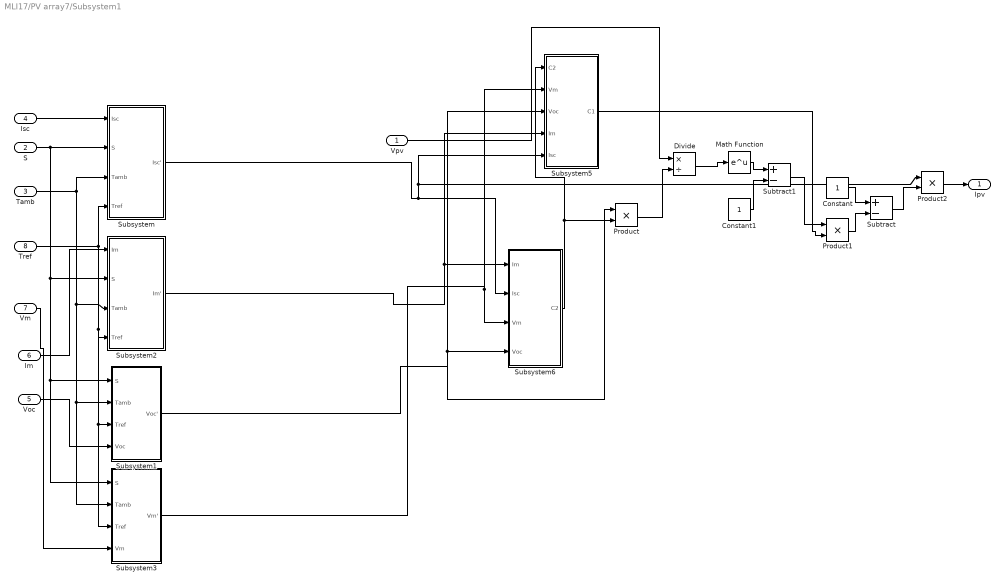
== system MLI17/PV array7/Subsystem1 ==
  Vpv : Inport
  S : Inport  Port=2
  Tamb : Inport  Port=3
  Isc : Inport  Port=4
  Voc : Inport  Port=5
  Im : Inport  Port=6
  Vm : Inport  Port=7
  Tref : Inport  Port=8
  Constant : Constant
  Constant1 : Constant
  Divide : Product  Inputs=*/
  Math Function : Math  SignedPower=on
  Product : Product  RndMeth=Zero
  Product1 : Product  RndMeth=Zero
  Product2 : Product  RndMeth=Zero
  Subsystem : Subsystem
  Subsystem1 : Subsystem
  Subsystem2 : Subsystem
  Subsystem3 : Subsystem
  Subsystem5 : Subsystem
  Subsystem6 : Subsystem
  Subtract : Sum  Inputs=+-
  Subtract1 : Sum  Inputs=+-
  Ipv : Outport
  wires:
  Product/1 -> Divide/2
  Constant/1 -> Subtract/1
  Product1/1 -> Subtract/2
  Subtract/1 -> Product2/2
  Product2/1 -> Ipv/1
  Divide/1 -> Math Function/1
  Math Function/1 -> Subtract1/1
  Constant1/1 -> Subtract1/2
  Subtract1/1 -> Product1/1
  Subsystem2/1(Im') -> Subsystem6/1(Im), Subsystem5/4(Im)
  Subsystem/1(Isc') -> Subsystem6/2(Isc), Product2/1, Subsystem5/5(Isc)
  Subsystem1/1(Voc') -> Product/1, Subsystem5/3(Voc), Subsystem6/4(Voc)
  Subsystem3/1(Vm') -> Subsystem5/2(Vm), Subsystem6/3(Vm)
  Subsystem6/1(C2) -> Subsystem5/1(C2), Product/2
  Vpv/1 -> Divide/1
  Subsystem5/1(C1) -> Product1/2
  Isc/1 -> Subsystem/1(Isc)
  S/1 -> Subsystem1/1(S), Subsystem3/1(S), Subsystem2/2(S), Subsystem/2(S)
  Tamb/1 -> Subsystem1/2(Tamb), Subsystem3/2(Tamb), Subsystem2/3(Tamb), Subsystem/3(Tamb)
  Tref/1 -> Subsystem1/3(Tref), Subsystem3/3(Tref), Subsystem2/4(Tref), Subsystem/4(Tref)
  Im/1 -> Subsystem2/1(Im)
  Voc/1 -> Subsystem1/4(Voc)
  Vm/1 -> Subsystem3/4(Vm)

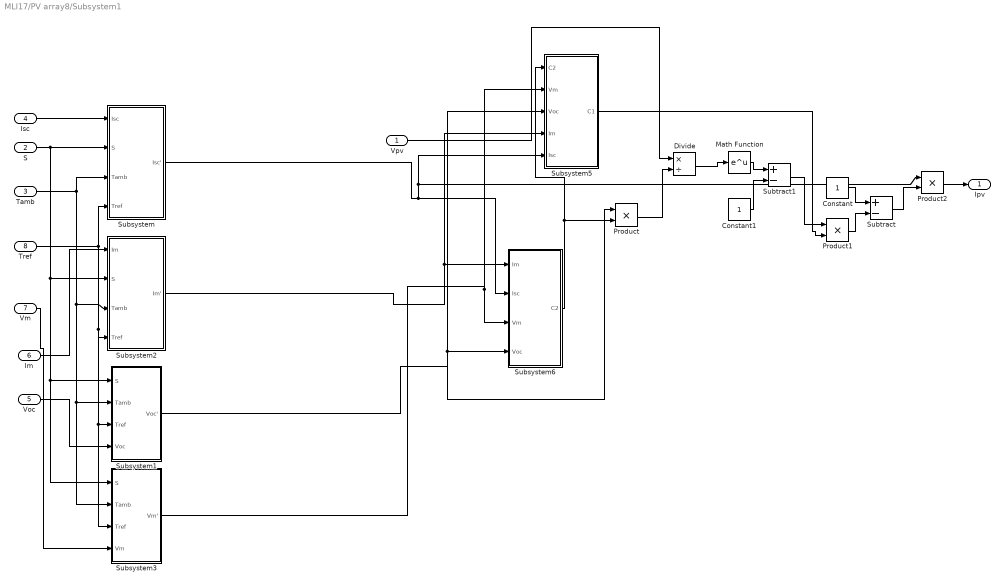
== system MLI17/PV array8/Subsystem1 ==
  Vpv : Inport
  S : Inport  Port=2
  Tamb : Inport  Port=3
  Isc : Inport  Port=4
  Voc : Inport  Port=5
  Im : Inport  Port=6
  Vm : Inport  Port=7
  Tref : Inport  Port=8
  Constant : Constant
  Constant1 : Constant
  Divide : Product  Inputs=*/
  Math Function : Math  SignedPower=on
  Product : Product  RndMeth=Zero
  Product1 : Product  RndMeth=Zero
  Product2 : Product  RndMeth=Zero
  Subsystem : Subsystem
  Subsystem1 : Subsystem
  Subsystem2 : Subsystem
  Subsystem3 : Subsystem
  Subsystem5 : Subsystem
  Subsystem6 : Subsystem
  Subtract : Sum  Inputs=+-
  Subtract1 : Sum  Inputs=+-
  Ipv : Outport
  wires:
  Vm/1 -> Subsystem3/4(Vm)
  Voc/1 -> Subsystem1/4(Voc)
  Im/1 -> Subsystem2/1(Im)
  Tref/1 -> Subsystem/4(Tref), Subsystem2/4(Tref), Subsystem3/3(Tref), Subsystem1/3(Tref)
  Tamb/1 -> Subsystem/3(Tamb), Subsystem2/3(Tamb), Subsystem3/2(Tamb), Subsystem1/2(Tamb)
  S/1 -> Subsystem/2(S), Subsystem2/2(S), Subsystem3/1(S), Subsystem1/1(S)
  Isc/1 -> Subsystem/1(Isc)
  Subsystem5/1(C1) -> Product1/2
  Vpv/1 -> Divide/1
  Subsystem6/1(C2) -> Product/2, Subsystem5/1(C2)
  Subsystem3/1(Vm') -> Subsystem6/3(Vm), Subsystem5/2(Vm)
  Subsystem1/1(Voc') -> Subsystem6/4(Voc), Subsystem5/3(Voc), Product/1
  Subsystem/1(Isc') -> Subsystem5/5(Isc), Product2/1, Subsystem6/2(Isc)
  Subsystem2/1(Im') -> Subsystem5/4(Im), Subsystem6/1(Im)
  Subtract1/1 -> Product1/1
  Constant1/1 -> Subtract1/2
  Math Function/1 -> Subtract1/1
  Divide/1 -> Math Function/1
  Product2/1 -> Ipv/1
  Subtract/1 -> Product2/2
  Product1/1 -> Subtract/2
  Constant/1 -> Subtract/1
  Product/1 -> Divide/2

== system MLI17/PV array1/Subsystem1/Subsystem ==
  Isc : Inport
  S : Inport  Port=2
  Tamb : Inport  Port=3
  Tref : Inport  Port=4
  Add : Sum
  Add1 : Sum
  Constant1 : Constant
  Constant2 : Constant  Value=0.03
  Divide : Product  Inputs=*/
  Product{,1..3} (4 alike) : Product  RndMeth=Zero
  Sref : Constant  Value=1000
  Subtract : Sum  Inputs=+-
  a : Constant  Value=0.0025
  Isc' : Outport
  wires:
  Subtract/1 -> Product/2
  a/1 -> Product/1
  Constant1/1 -> Add/2
  Product/1 -> Add/1
  Isc/1 -> Product1/1
  S/1 -> Product1/2, Product3/1
  Product1/1 -> Product2/1
  Add/1 -> Product2/2
  Product2/1 -> Divide/1
  Sref/1 -> Divide/2
  Divide/1 -> Isc'/1
  Tref/1 -> Subtract/2
  Constant2/1 -> Product3/2
  Product3/1 -> Add1/1
  Tamb/1 -> Add1/2
  Add1/1 -> Subtract/1

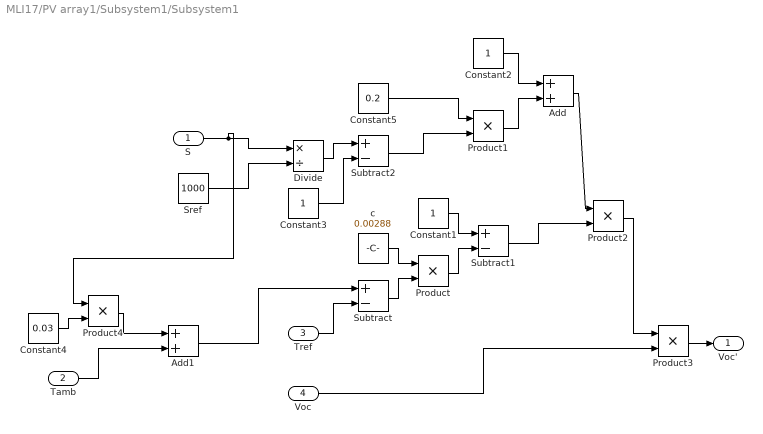
== system MLI17/PV array1/Subsystem1/Subsystem1 ==
  S : Inport
  Tamb : Inport  Port=2
  Tref : Inport  Port=3
  Voc : Inport  Port=4
  Add : Sum
  Add1 : Sum
  Constant1 : Constant
  Constant2 : Constant
  Constant3 : Constant
  Constant4 : Constant  Value=0.03
  Constant5 : Constant  Value=0.2
  Divide : Product  Inputs=*/
  Product{,1..4} (5 alike) : Product  RndMeth=Zero
  Sref : Constant  Value=1000
  Subtract : Sum  Inputs=+-
  Subtract1 : Sum  Inputs=+-
  Subtract2 : Sum  Inputs=+-
  c : Constant  Value=0.00288
  Voc' : Outport
  wires:
  Tref/1 -> Subtract/2
  c/1 -> Product/1
  Subtract/1 -> Product/2
  Constant1/1 -> Subtract1/1
  Product/1 -> Subtract1/2
  Subtract2/1 -> Product1/2
  Constant2/1 -> Add/1
  Product1/1 -> Add/2
  Subtract1/1 -> Product2/2
  Add/1 -> Product2/1
  Product2/1 -> Product3/1
  Voc/1 -> Product3/2
  Product3/1 -> Voc'/1
  S/1 -> Divide/1, Product4/1
  Sref/1 -> Divide/2
  Divide/1 -> Subtract2/1
  Constant3/1 -> Subtract2/2
  Constant4/1 -> Product4/2
  Product4/1 -> Add1/1
  Tamb/1 -> Add1/2
  Add1/1 -> Subtract/1
  Constant5/1 -> Product1/1

== system MLI17/PV array1/Subsystem1/Subsystem2 ==
  Im : Inport
  S : Inport  Port=2
  Tamb : Inport  Port=3
  Tref : Inport  Port=4
  Add : Sum
  Add1 : Sum
  Constant1 : Constant
  Constant2 : Constant  Value=0.03
  Divide : Product  Inputs=*/
  Product{,1..3} (4 alike) : Product  RndMeth=Zero
  Sref : Constant  Value=1000
  Subtract : Sum  Inputs=+-
  a : Constant  Value=0.0025
  Im' : Outport
  wires:
  Subtract/1 -> Product/2
  a/1 -> Product/1
  Constant1/1 -> Add/2
  Product/1 -> Add/1
  Im/1 -> Product1/1
  S/1 -> Product1/2, Product3/1
  Product1/1 -> Product2/1
  Add/1 -> Product2/2
  Product2/1 -> Divide/1
  Sref/1 -> Divide/2
  Divide/1 -> Im'/1
  Tref/1 -> Subtract/2
  Constant2/1 -> Product3/2
  Product3/1 -> Add1/1
  Tamb/1 -> Add1/2
  Add1/1 -> Subtract/1

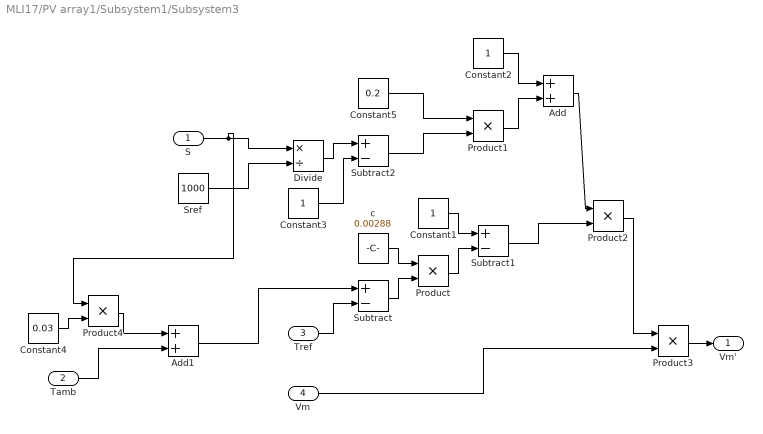
== system MLI17/PV array1/Subsystem1/Subsystem3 ==
  S : Inport
  Tamb : Inport  Port=2
  Tref : Inport  Port=3
  Vm : Inport  Port=4
  Add : Sum
  Add1 : Sum
  Constant1 : Constant
  Constant2 : Constant
  Constant3 : Constant
  Constant4 : Constant  Value=0.03
  Constant5 : Constant  Value=0.2
  Divide : Product  Inputs=*/
  Product{,1..4} (5 alike) : Product  RndMeth=Zero
  Sref : Constant  Value=1000
  Subtract : Sum  Inputs=+-
  Subtract1 : Sum  Inputs=+-
  Subtract2 : Sum  Inputs=+-
  c : Constant  Value=0.00288
  Vm' : Outport
  wires:
  Tref/1 -> Subtract/2
  c/1 -> Product/1
  Subtract/1 -> Product/2
  Constant1/1 -> Subtract1/1
  Product/1 -> Subtract1/2
  Subtract2/1 -> Product1/2
  Constant2/1 -> Add/1
  Product1/1 -> Add/2
  Subtract1/1 -> Product2/2
  Add/1 -> Product2/1
  Product2/1 -> Product3/1
  Vm/1 -> Product3/2
  Product3/1 -> Vm'/1
  S/1 -> Divide/1, Product4/1
  Sref/1 -> Divide/2
  Divide/1 -> Subtract2/1
  Constant3/1 -> Subtract2/2
  Constant4/1 -> Product4/2
  Product4/1 -> Add1/1
  Tamb/1 -> Add1/2
  Add1/1 -> Subtract/1
  Constant5/1 -> Product1/1

== system MLI17/PV array1/Subsystem1/Subsystem5 ==
  C2 : Inport
  Vm : Inport  Port=2
  Voc : Inport  Port=3
  Im : Inport  Port=4
  Isc : Inport  Port=5
  Constant : Constant
  Constant1 : Constant  Value=-1
  Divide : Product  Inputs=*/
  Divide1 : Product  Inputs=*/
  Math Function : Math  SignedPower=on
  Product : Product  RndMeth=Zero
  Product1 : Product  RndMeth=Zero
  Product2 : Product  RndMeth=Zero
  Subtract : Sum  Inputs=+-
  C1 : Outport
  wires:
  Product/1 -> Divide1/2
  Divide1/1 -> Product1/2
  Constant1/1 -> Product1/1
  Product1/1 -> Math Function/1
  Math Function/1 -> Product2/1
  Subtract/1 -> Product2/2
  Product2/1 -> C1/1
  Vm/1 -> Divide1/1
  Voc/1 -> Product/2
  C2/1 -> Product/1
  Im/1 -> Divide/1
  Isc/1 -> Divide/2
  Constant/1 -> Subtract/1
  Divide/1 -> Subtract/2

== system MLI17/PV array1/Subsystem1/Subsystem6 ==
  Im : Inport
  Isc : Inport  Port=2
  Vm : Inport  Port=3
  Voc : Inport  Port=4
  Constant : Constant
  Constant1 : Constant
  Divide : Product  Inputs=*/
  Divide1 : Product  Inputs=*/
  Divide2 : Product  Inputs=*/
  Math Function : Math  Operator=log  SignedPower=on
  Subtract : Sum  Inputs=+-
  Subtract1 : Sum  Inputs=+-
  C2 : Outport
  wires:
  Divide/1 -> Subtract/1
  Constant/1 -> Subtract/2
  Constant1/1 -> Subtract1/1
  Divide1/1 -> Subtract1/2
  Divide2/1 -> C2/1
  Vm/1 -> Divide/1
  Voc/1 -> Divide/2
  Im/1 -> Divide1/1
  Isc/1 -> Divide1/2
  Subtract1/1 -> Math Function/1
  Subtract/1 -> Divide2/1
  Math Function/1 -> Divide2/2

== system MLI17/PV array2/Subsystem1/Subsystem ==
  Isc : Inport
  S : Inport  Port=2
  Tamb : Inport  Port=3
  Tref : Inport  Port=4
  Add : Sum
  Add1 : Sum
  Constant1 : Constant
  Constant2 : Constant  Value=0.03
  Divide : Product  Inputs=*/
  Product{,1..3} (4 alike) : Product  RndMeth=Zero
  Sref : Constant  Value=1000
  Subtract : Sum  Inputs=+-
  a : Constant  Value=0.0025
  Isc' : Outport
  wires:
  Add1/1 -> Subtract/1
  Tamb/1 -> Add1/2
  Product3/1 -> Add1/1
  Constant2/1 -> Product3/2
  Tref/1 -> Subtract/2
  Divide/1 -> Isc'/1
  Sref/1 -> Divide/2
  Product2/1 -> Divide/1
  Add/1 -> Product2/2
  Product1/1 -> Product2/1
  S/1 -> Product3/1, Product1/2
  Isc/1 -> Product1/1
  Product/1 -> Add/1
  Constant1/1 -> Add/2
  a/1 -> Product/1
  Subtract/1 -> Product/2

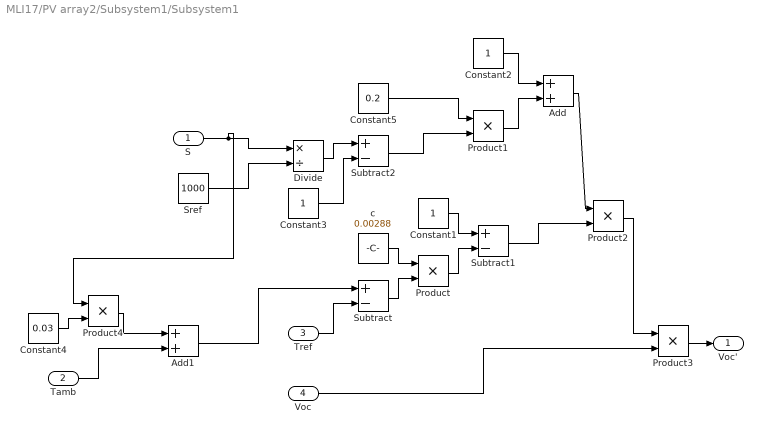
== system MLI17/PV array2/Subsystem1/Subsystem1 ==
  S : Inport
  Tamb : Inport  Port=2
  Tref : Inport  Port=3
  Voc : Inport  Port=4
  Add : Sum
  Add1 : Sum
  Constant1 : Constant
  Constant2 : Constant
  Constant3 : Constant
  Constant4 : Constant  Value=0.03
  Constant5 : Constant  Value=0.2
  Divide : Product  Inputs=*/
  Product{,1..4} (5 alike) : Product  RndMeth=Zero
  Sref : Constant  Value=1000
  Subtract : Sum  Inputs=+-
  Subtract1 : Sum  Inputs=+-
  Subtract2 : Sum  Inputs=+-
  c : Constant  Value=0.00288
  Voc' : Outport
  wires:
  Constant5/1 -> Product1/1
  Add1/1 -> Subtract/1
  Tamb/1 -> Add1/2
  Product4/1 -> Add1/1
  Constant4/1 -> Product4/2
  Constant3/1 -> Subtract2/2
  Divide/1 -> Subtract2/1
  Sref/1 -> Divide/2
  S/1 -> Product4/1, Divide/1
  Product3/1 -> Voc'/1
  Voc/1 -> Product3/2
  Product2/1 -> Product3/1
  Add/1 -> Product2/1
  Subtract1/1 -> Product2/2
  Product1/1 -> Add/2
  Constant2/1 -> Add/1
  Subtract2/1 -> Product1/2
  Product/1 -> Subtract1/2
  Constant1/1 -> Subtract1/1
  Subtract/1 -> Product/2
  c/1 -> Product/1
  Tref/1 -> Subtract/2

== system MLI17/PV array2/Subsystem1/Subsystem2 ==
  Im : Inport
  S : Inport  Port=2
  Tamb : Inport  Port=3
  Tref : Inport  Port=4
  Add : Sum
  Add1 : Sum
  Constant1 : Constant
  Constant2 : Constant  Value=0.03
  Divide : Product  Inputs=*/
  Product{,1..3} (4 alike) : Product  RndMeth=Zero
  Sref : Constant  Value=1000
  Subtract : Sum  Inputs=+-
  a : Constant  Value=0.0025
  Im' : Outport
  wires:
  Add1/1 -> Subtract/1
  Tamb/1 -> Add1/2
  Product3/1 -> Add1/1
  Constant2/1 -> Product3/2
  Tref/1 -> Subtract/2
  Divide/1 -> Im'/1
  Sref/1 -> Divide/2
  Product2/1 -> Divide/1
  Add/1 -> Product2/2
  Product1/1 -> Product2/1
  S/1 -> Product3/1, Product1/2
  Im/1 -> Product1/1
  Product/1 -> Add/1
  Constant1/1 -> Add/2
  a/1 -> Product/1
  Subtract/1 -> Product/2

== system MLI17/PV array2/Subsystem1/Subsystem3 ==
  S : Inport
  Tamb : Inport  Port=2
  Tref : Inport  Port=3
  Vm : Inport  Port=4
  Add : Sum
  Add1 : Sum
  Constant1 : Constant
  Constant2 : Constant
  Constant3 : Constant
  Constant4 : Constant  Value=0.03
  Constant5 : Constant  Value=0.2
  Divide : Product  Inputs=*/
  Product{,1..4} (5 alike) : Product  RndMeth=Zero
  Sref : Constant  Value=1000
  Subtract : Sum  Inputs=+-
  Subtract1 : Sum  Inputs=+-
  Subtract2 : Sum  Inputs=+-
  c : Constant  Value=0.00288
  Vm' : Outport
  wires:
  Constant5/1 -> Product1/1
  Add1/1 -> Subtract/1
  Tamb/1 -> Add1/2
  Product4/1 -> Add1/1
  Constant4/1 -> Product4/2
  Constant3/1 -> Subtract2/2
  Divide/1 -> Subtract2/1
  Sref/1 -> Divide/2
  S/1 -> Product4/1, Divide/1
  Product3/1 -> Vm'/1
  Vm/1 -> Product3/2
  Product2/1 -> Product3/1
  Add/1 -> Product2/1
  Subtract1/1 -> Product2/2
  Product1/1 -> Add/2
  Constant2/1 -> Add/1
  Subtract2/1 -> Product1/2
  Product/1 -> Subtract1/2
  Constant1/1 -> Subtract1/1
  Subtract/1 -> Product/2
  c/1 -> Product/1
  Tref/1 -> Subtract/2

== system MLI17/PV array2/Subsystem1/Subsystem5 ==
  C2 : Inport
  Vm : Inport  Port=2
  Voc : Inport  Port=3
  Im : Inport  Port=4
  Isc : Inport  Port=5
  Constant : Constant
  Constant1 : Constant  Value=-1
  Divide : Product  Inputs=*/
  Divide1 : Product  Inputs=*/
  Math Function : Math  SignedPower=on
  Product : Product  RndMeth=Zero
  Product1 : Product  RndMeth=Zero
  Product2 : Product  RndMeth=Zero
  Subtract : Sum  Inputs=+-
  C1 : Outport
  wires:
  Divide/1 -> Subtract/2
  Constant/1 -> Subtract/1
  Isc/1 -> Divide/2
  Im/1 -> Divide/1
  C2/1 -> Product/1
  Voc/1 -> Product/2
  Vm/1 -> Divide1/1
  Product2/1 -> C1/1
  Subtract/1 -> Product2/2
  Math Function/1 -> Product2/1
  Product1/1 -> Math Function/1
  Constant1/1 -> Product1/1
  Divide1/1 -> Product1/2
  Product/1 -> Divide1/2

== system MLI17/PV array2/Subsystem1/Subsystem6 ==
  Im : Inport
  Isc : Inport  Port=2
  Vm : Inport  Port=3
  Voc : Inport  Port=4
  Constant : Constant
  Constant1 : Constant
  Divide : Product  Inputs=*/
  Divide1 : Product  Inputs=*/
  Divide2 : Product  Inputs=*/
  Math Function : Math  Operator=log  SignedPower=on
  Subtract : Sum  Inputs=+-
  Subtract1 : Sum  Inputs=+-
  C2 : Outport
  wires:
  Math Function/1 -> Divide2/2
  Subtract/1 -> Divide2/1
  Subtract1/1 -> Math Function/1
  Isc/1 -> Divide1/2
  Im/1 -> Divide1/1
  Voc/1 -> Divide/2
  Vm/1 -> Divide/1
  Divide2/1 -> C2/1
  Divide1/1 -> Subtract1/2
  Constant1/1 -> Subtract1/1
  Constant/1 -> Subtract/2
  Divide/1 -> Subtract/1

== system MLI17/PV array3/Subsystem1/Subsystem ==
  Isc : Inport
  S : Inport  Port=2
  Tamb : Inport  Port=3
  Tref : Inport  Port=4
  Add : Sum
  Add1 : Sum
  Constant1 : Constant
  Constant2 : Constant  Value=0.03
  Divide : Product  Inputs=*/
  Product{,1..3} (4 alike) : Product  RndMeth=Zero
  Sref : Constant  Value=1000
  Subtract : Sum  Inputs=+-
  a : Constant  Value=0.0025
  Isc' : Outport
  wires:
  Subtract/1 -> Product/2
  a/1 -> Product/1
  Constant1/1 -> Add/2
  Product/1 -> Add/1
  Isc/1 -> Product1/1
  S/1 -> Product1/2, Product3/1
  Product1/1 -> Product2/1
  Add/1 -> Product2/2
  Product2/1 -> Divide/1
  Sref/1 -> Divide/2
  Divide/1 -> Isc'/1
  Tref/1 -> Subtract/2
  Constant2/1 -> Product3/2
  Product3/1 -> Add1/1
  Tamb/1 -> Add1/2
  Add1/1 -> Subtract/1

== system MLI17/PV array3/Subsystem1/Subsystem1 ==
  S : Inport
  Tamb : Inport  Port=2
  Tref : Inport  Port=3
  Voc : Inport  Port=4
  Add : Sum
  Add1 : Sum
  Constant1 : Constant
  Constant2 : Constant
  Constant3 : Constant
  Constant4 : Constant  Value=0.03
  Constant5 : Constant  Value=0.2
  Divide : Product  Inputs=*/
  Product{,1..4} (5 alike) : Product  RndMeth=Zero
  Sref : Constant  Value=1000
  Subtract : Sum  Inputs=+-
  Subtract1 : Sum  Inputs=+-
  Subtract2 : Sum  Inputs=+-
  c : Constant  Value=0.00288
  Voc' : Outport
  wires:
  Tref/1 -> Subtract/2
  c/1 -> Product/1
  Subtract/1 -> Product/2
  Constant1/1 -> Subtract1/1
  Product/1 -> Subtract1/2
  Subtract2/1 -> Product1/2
  Constant2/1 -> Add/1
  Product1/1 -> Add/2
  Subtract1/1 -> Product2/2
  Add/1 -> Product2/1
  Product2/1 -> Product3/1
  Voc/1 -> Product3/2
  Product3/1 -> Voc'/1
  S/1 -> Divide/1, Product4/1
  Sref/1 -> Divide/2
  Divide/1 -> Subtract2/1
  Constant3/1 -> Subtract2/2
  Constant4/1 -> Product4/2
  Product4/1 -> Add1/1
  Tamb/1 -> Add1/2
  Add1/1 -> Subtract/1
  Constant5/1 -> Product1/1

== system MLI17/PV array3/Subsystem1/Subsystem2 ==
  Im : Inport
  S : Inport  Port=2
  Tamb : Inport  Port=3
  Tref : Inport  Port=4
  Add : Sum
  Add1 : Sum
  Constant1 : Constant
  Constant2 : Constant  Value=0.03
  Divide : Product  Inputs=*/
  Product{,1..3} (4 alike) : Product  RndMeth=Zero
  Sref : Constant  Value=1000
  Subtract : Sum  Inputs=+-
  a : Constant  Value=0.0025
  Im' : Outport
  wires:
  Subtract/1 -> Product/2
  a/1 -> Product/1
  Constant1/1 -> Add/2
  Product/1 -> Add/1
  Im/1 -> Product1/1
  S/1 -> Product1/2, Product3/1
  Product1/1 -> Product2/1
  Add/1 -> Product2/2
  Product2/1 -> Divide/1
  Sref/1 -> Divide/2
  Divide/1 -> Im'/1
  Tref/1 -> Subtract/2
  Constant2/1 -> Product3/2
  Product3/1 -> Add1/1
  Tamb/1 -> Add1/2
  Add1/1 -> Subtract/1

== system MLI17/PV array3/Subsystem1/Subsystem3 ==
  S : Inport
  Tamb : Inport  Port=2
  Tref : Inport  Port=3
  Vm : Inport  Port=4
  Add : Sum
  Add1 : Sum
  Constant1 : Constant
  Constant2 : Constant
  Constant3 : Constant
  Constant4 : Constant  Value=0.03
  Constant5 : Constant  Value=0.2
  Divide : Product  Inputs=*/
  Product{,1..4} (5 alike) : Product  RndMeth=Zero
  Sref : Constant  Value=1000
  Subtract : Sum  Inputs=+-
  Subtract1 : Sum  Inputs=+-
  Subtract2 : Sum  Inputs=+-
  c : Constant  Value=0.00288
  Vm' : Outport
  wires:
  Tref/1 -> Subtract/2
  c/1 -> Product/1
  Subtract/1 -> Product/2
  Constant1/1 -> Subtract1/1
  Product/1 -> Subtract1/2
  Subtract2/1 -> Product1/2
  Constant2/1 -> Add/1
  Product1/1 -> Add/2
  Subtract1/1 -> Product2/2
  Add/1 -> Product2/1
  Product2/1 -> Product3/1
  Vm/1 -> Product3/2
  Product3/1 -> Vm'/1
  S/1 -> Divide/1, Product4/1
  Sref/1 -> Divide/2
  Divide/1 -> Subtract2/1
  Constant3/1 -> Subtract2/2
  Constant4/1 -> Product4/2
  Product4/1 -> Add1/1
  Tamb/1 -> Add1/2
  Add1/1 -> Subtract/1
  Constant5/1 -> Product1/1

== system MLI17/PV array3/Subsystem1/Subsystem5 ==
  C2 : Inport
  Vm : Inport  Port=2
  Voc : Inport  Port=3
  Im : Inport  Port=4
  Isc : Inport  Port=5
  Constant : Constant
  Constant1 : Constant  Value=-1
  Divide : Product  Inputs=*/
  Divide1 : Product  Inputs=*/
  Math Function : Math  SignedPower=on
  Product : Product  RndMeth=Zero
  Product1 : Product  RndMeth=Zero
  Product2 : Product  RndMeth=Zero
  Subtract : Sum  Inputs=+-
  C1 : Outport
  wires:
  Product/1 -> Divide1/2
  Divide1/1 -> Product1/2
  Constant1/1 -> Product1/1
  Product1/1 -> Math Function/1
  Math Function/1 -> Product2/1
  Subtract/1 -> Product2/2
  Product2/1 -> C1/1
  Vm/1 -> Divide1/1
  Voc/1 -> Product/2
  C2/1 -> Product/1
  Im/1 -> Divide/1
  Isc/1 -> Divide/2
  Constant/1 -> Subtract/1
  Divide/1 -> Subtract/2

== system MLI17/PV array3/Subsystem1/Subsystem6 ==
  Im : Inport
  Isc : Inport  Port=2
  Vm : Inport  Port=3
  Voc : Inport  Port=4
  Constant : Constant
  Constant1 : Constant
  Divide : Product  Inputs=*/
  Divide1 : Product  Inputs=*/
  Divide2 : Product  Inputs=*/
  Math Function : Math  Operator=log  SignedPower=on
  Subtract : Sum  Inputs=+-
  Subtract1 : Sum  Inputs=+-
  C2 : Outport
  wires:
  Divide/1 -> Subtract/1
  Constant/1 -> Subtract/2
  Constant1/1 -> Subtract1/1
  Divide1/1 -> Subtract1/2
  Divide2/1 -> C2/1
  Vm/1 -> Divide/1
  Voc/1 -> Divide/2
  Im/1 -> Divide1/1
  Isc/1 -> Divide1/2
  Subtract1/1 -> Math Function/1
  Subtract/1 -> Divide2/1
  Math Function/1 -> Divide2/2
